simulink model "final_gimbal"  (R2026b)
settings: Solver=ode23t  StopTime=10  MaxStep=max_step  RelTol=1e-4
values from neighbouring files (symbols this model uses):
  kg = SV(i,7)    [servo_dynamics.m]
  m = add_block('simulink/Signal Routing/Mux', sprintf('    [build_model.m]
  N = 0    [LiveView.m]
  s = (1 - a) * B(k, 2:7) + a * B(k+1, 2:7)    [UdpAttitudeSource.m]    (also in build_model.m = solid(mdl, name, 'servo_dummy.stl', color, pos + [90 0 90 0])
  stl = fullfile(fileparts(fileparts(mfilename('fullpath'))), 'cad', 'stl')    [LiveView.m]
undefined symbols (not defined in the file or in its folder): ant_mass, lead_s, log_dt, mount_rate, pwm_rate, q0, servo_mass, SV, t_pure, travel, X, Y, Z
libraries: sm_lib x67, nesl_utility x18
(part 2 of 2)

== matlab function final_gimbal/servo ==
  data: cmd input; tgear output; q input; qd input; qm input; qmd input; SV input; qmdd output; sat output
function [tgear, qmdd, sat] = f(cmd, q, qd, qm, qmd, SV)
[tgear, qmdd, sat] = servo_dynamics(cmd, q, qd, qm, qmd, SV);

== matlab function final_gimbal/antenna_angles ==
  data: R input; ant output
function ant = f(R)
% antenna roll, pitch (flight-controller convention: nose up +) and total tilt [deg]
R = reshape(R, 3, 3);
ant = [atan2(R(3,2), R(3,3)); asin(max(-1, min(1, R(3,1)))); acos(max(-1, min(1, R(3,3))))] * 180/pi;
